simulink model "QDrone_Capture_IMU"  (R2019a)
settings: Solver=ode2  StartTime=0.0  StopTime=inf  FixedStep=0.001  RelTol=1e-3  EnableMultiTasking=on
InitFcn:
  | addpath(fullfile(fileparts(get_param('QDrone_Capture_IMU','FileName')),'capture_tool'));
model workspace (MAT data in the model file):
  target_system = 1
undefined symbols (not defined in the file or in its folder): HIL, qc_get_step_size
libraries: quarc_library x7
settings Model: SimulationMode=external  ExtModeTrigDuration=10000  Creator=dmadill  LastModifiedBy=user
settings SolverCC: PositivePriorityOrder=on
settings DataIOCC: LimitDataPoints=on  SaveFormat=Array  ReturnWorkspaceOutputs=off
settings OptimizationCC: LifeSpan=inf
settings DebuggingCC: SolverPrmCheckMsg=warning  SFUnexpectedBacktrackingDiag=warning  SFNoUnconditionalDefaultTransitionDiag=warning  SFExecutionAtInitializationDiag=none  ArithmeticOperatorsInVariantConditions=warning
settings HardwareCC: ProdBitPerLong=64  ProdLargestAtomicFloat=None  ProdHWDeviceType=Intel->x86-64
settings ModelReferenceCC: PropagateSignalLabelsOutOfModel=off
settings SFSimCC: SimUseLocalCustomCode=off
settings RTWCC: SystemTargetFile=quarc_linux_x64.tlc  TemplateMakefile=quarc_linux_x64_tmf  Description=QUARC Linux x64 Target  RTWUseLocalCustomCode=off
settings CodeAppCC: StateflowObjectComments=on
settings STFCustomTargetCC: TargetLibSuffix=.a  TargetPreCompLibLocation=C:\PROGRA~3\QUARC\lib\2019a\LINUX_~1\release  ConcurrentExecutionCompliant=on  SystemTargetFile=quarc_linux_x64.tlc
settings GRTTargetCC: TargetLibSuffix=.a  TargetPreCompLibLocation=C:\PROGRA~3\QUARC\lib\2019a\LINUX_~1\release  TargetLangStandard=C89/C90 (ANSI)  ParMdlRefBuildCompliant=off  CompOptLevelCompliant=off  CombineOutputUpdateFcns=off  MatFileLogging=off  CPPClassGenCompliant=off  GRTInterface=on  UseToolchainInfoCompliant=off  ExtMode=on  ExtModeMexFile=quarc_comm  ExtModeMexArgs='-w -d /tmp -uri %u', 'tcpip://192.168.2.52:17001?retries=10', 'tcpip://192.168.2.52:17000'
settings ConfigComp: CovMetricSettings=dw  CovHtmlReporting=on  CovSaveCumulativeToWorkspaceVar=on  CovSaveSingleToWorkspaceVar=on  CovExternalEMLEnable=off  CovSFcnEnable=off

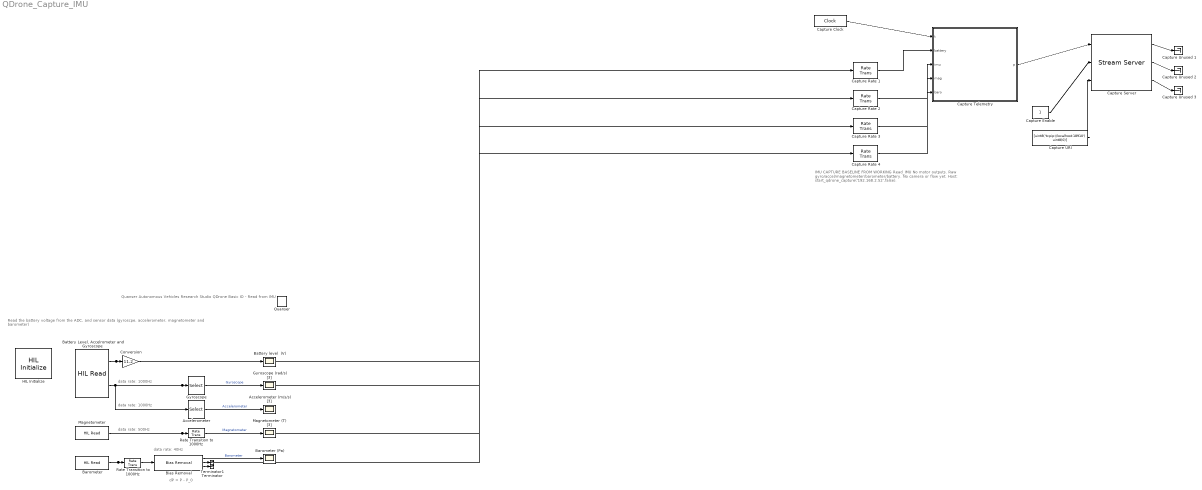
== system QDrone_Capture_IMU ==
  note: Quanser Autonomous Vehicles Research Studio
      | QDrone Basic IO - Read from IMU
  note: Read the battery voltage from the ADC, and sensor data (gyroscpe, accelerometer, magnetometer and barometer)
  note: data rate: 40Hz
  note: dP = P - P_0
  note: data rate: 500Hz
  note: data rate: 1000Hz
  note: data rate: 1000Hz
  note: IMU CAPTURE BASELINE FROM WORKING Read_IMU
      | No motor outputs. Raw gyro/accel/magnetometer/barometer/battery.
      | No camera or flow yet. Host: start_qdrone_capture('192.168.2.52',false).
  Accelerometer : Selector  InputPortWidth=6  IndexOptions=Index vector (dialog)  Indices=[4:6]  OutputSizes=1
  Accelerometer (m/s/s) [3] : Scope
  Barometer : quarc_library/Data Acquisition/Generic/Immediate I//O/HIL Read  Priority=1  object_name=HIL-1  analog_channels=[]  encoder_channels=[]  digital_channels=[]  other_channels=[9000]  sample_time=qc_get_step_size*25  active=on  vector_output=on  data_type_mode=Inherit via back propagation  encoder_data_type=double  digital_data_type=boolean
      settings: SourceProductName=The database C:\Users\user\AppData\Roaming\MathWorks\MATLAB\R2017a\slblocks_master.db is locked, or a table in the database is locked. (database is locked)
  Barometer (Pa) : Scope
  "Battery Level, Accelrometer and Gyroscope" : quarc_library/Data Acquisition/Generic/Immediate I//O/HIL Read  Priority=1  object_name=HIL-1  analog_channels=[4]  encoder_channels=[]  digital_channels=[]  other_channels=[3000:3002 4000:4002]  sample_time=qc_get_step_size  active=on  vector_output=on  data_type_mode=Inherit via back propagation  encoder_data_type=double  digital_data_type=boolean
      settings: SourceProductName=The database C:\Users\user\AppData\Roaming\MathWorks\MATLAB\R2017a\slblocks_master.db is locked, or a table in the database is locked. (database is locked)
  Battery level  (V) : Scope
  Bias Removal : quarc_library/Discrete/Bias Removal  start_time=0  end_time=2  switch_id=X  sample_time=qc_get_step_size
      settings: SourceProductName=QUARC Targets
  Capture Clock : DigitalClock  SampleTime=0.001
  Capture Enable : Constant
  Capture Rate {1..4} (4 alike) : RateTransition  OutPortSampleTime=0.001
  Capture Server : quarc_library/Communications/Basic/Stream Server  uri_source=External input port  uri=tcpip://remotehost:18000  apply_uri_to_all_configs=on  send_buffer_size=65536  receive_buffer_size=1024  byte_order=little endian (Intel - LSB first)  optimization=Minimum latency  send_options=Send all data  receive_options=Do not receive data  default_value=[0]  sample_time=0.001  active=on  implementation=Use blocking I/O in a separate thread  send_fifo_size=20000  receive_fifo_size=1000  send_priority=0  receive_priority=0  send_dimensions=off  receive_dimensions=off  max_dimensions=-1  data_type=Inherited via back propagation  type_expr=BusObject
  Capture Telemetry : MATLAB Function  TreatAsAtomicUnit=on
  Capture URI : Constant  Value=[uint8('tcpip://localhost:18910') uint8(0)]
  Capture Unused 1 : Terminator
  Capture Unused 2 : Terminator
  Capture Unused 3 : Terminator
  Conversion : Gain  Gain=11.2
  Gyroscope : Selector  InputPortWidth=6  IndexOptions=Index vector (dialog)  Indices=[1:3]  OutputSizes=1
  Gyroscope (rad/s) [3] : Scope
  HIL Initialize : quarc_library/Data Acquisition/Generic/Configuration/HIL Initialize  object_name=HIL-1  board_type=qdrone  board_number=0  board_options=gyro_fs=2000;gyro_rate=1000;gyro_os=4;accel_fs=16;accel_rate=400;accel_os=4;baro_os=4096  exclusive=off  active=on  hardware_clocks=[]  clock_modes=[]  initial_clock_frequencies=[]  set_clock_params_at_start=off  set_clock_params_at_switch_in=off  set_clock_frequencies_at_start=off  set_clock_frequencies_at_switch_in=off  analog_input_channels=[0:4]  analog_input_configurations=[]  analog_input_maximums=[3.3]  analog_input_minimums=[0]  set_analog_input_params_at_start=off  set_analog_input_params_at_switch_in=off  analog_output_channels=[]  analog_output_maximums=[]  analog_output_minimums=[]  initial_analog_outputs=[]  final_analog_outputs=[]  watchdog_analog_outputs=[]  set_analog_output_params_at_start=off  set_analog_output_params_at_switch_in=off  set_analog_outputs_at_start=off  set_analog_outputs_at_switch_in=off  set_analog_outputs_at_terminate=off  set_analog_outputs_at_switch_out=off  set_analog_outputs_on_watchdog=off  digital_input_channels=[]  digital_output_channels=[]  digital_output_configuration=[]  initial_digital_outputs=[0]  final_digital_outputs=[0]  watchdog_digital_outputs=[]  set_digital_output_params_at_start=off  set_digital_output_params_at_switch_in=off  set_digital_outputs_at_start=off  set_digital_outputs_at_switch_in=off  set_digital_outputs_at_terminate=off  set_digital_outputs_at_switch_out=off  set_digital_outputs_on_watchdog=off  encoder_channels=[]  quadrature=[4]  encoder_filter_frequency=50e6/1  initial_encoder_counts=[0]  set_encoder_params_at_start=off  set_encoder_params_at_switch_in=off  set_encoder_counts_at_start=off  set_encoder_counts_at_switch_in=off  pwm_channels=[]  pwm_modes=[4]  pwm_frequency=2000  pwm_configuration=[0]  pwm_alignment=[0]  pwm_polarity=[1]  pwm_leading_deadband=[]  pwm_trailing_deadband=[]  initial_pwm_outputs=[0]  final_pwm_outputs=[0]  watchdog_pwm_outputs=[0]  set_pwm_params_at_start=off  set_pwm_params_at_switch_in=off  set_pwm_outputs_at_start=off  set_pwm_outputs_at_switch_in=off  set_pwm_outputs_at_terminate=off  set_pwm_outputs_at_switch_out=off  set_pwm_outputs_on_watchdog=off  other_output_channels=[]  initial_other_outputs=[]  final_other_outputs=[]  watchdog_other_outputs=[]  set_other_outputs_at_start=off  set_other_outputs_at_switch_in=off  set_other_outputs_at_terminate=off  set_other_outputs_at_switch_out=off  set_other_outputs_on_watchdog=off
      settings: SourceProductName=The database C:\Users\user\AppData\Roaming\MathWorks\MATLAB\R2017a\slblocks_master.db is locked, or a table in the database is locked. (database is locked)
  Magnetometer : quarc_library/Data Acquisition/Generic/Immediate I//O/HIL Read  Priority=1  object_name=HIL-1  analog_channels=[]  encoder_channels=[]  digital_channels=[]  other_channels=[8000:8002]  sample_time=qc_get_step_size*2  active=on  vector_output=on  data_type_mode=Inherit via back propagation  encoder_data_type=double  digital_data_type=boolean
      settings: SourceProductName=The database C:\Users\user\AppData\Roaming\MathWorks\MATLAB\R2017a\slblocks_master.db is locked, or a table in the database is locked. (database is locked)
  Magnetometer (T) [3] : Scope
  Quanser : quarc_library/Logos/Quanser
  Rate Transition to 1000Hz : RateTransition
  Rate Transition to 1000Hz : RateTransition  OutPortSampleTime=qc_get_step_size
  Terminator : Terminator
  Terminator1 : Terminator
  wires:
  Accelerometer/1 -> Accelerometer (m/s/s) [3]/1  "Accelerometer"
  Bias Removal/3 -> Terminator/1
  Gyroscope/1 -> Gyroscope (rad/s) [3]/1  "Gyroscope"
  Barometer/1 -> Rate Transition to 1000Hz/1, Capture Rate 4/1
  Bias Removal/1 -> Barometer (Pa)/1  "Barometer"
  "Battery Level, Accelrometer and Gyroscope"/1 -> Conversion/1, Capture Rate 1/1
  Bias Removal/2 -> Terminator1/1
  Magnetometer/1 -> Rate Transition to 1000Hz/1, Capture Rate 3/1
  Rate Transition to 1000Hz/1 -> Magnetometer (T) [3]/1  "Magnetometer"
  Conversion/1 -> Battery level  (V)/1
  "Battery Level, Accelrometer and Gyroscope"/2 -> Capture Rate 2/1, Gyroscope/1, Accelerometer/1
  Rate Transition to 1000Hz/1 -> Bias Removal/1
  Capture Clock/1 -> Capture Telemetry/1(t)
  Capture Rate 1/1 -> Capture Telemetry/2(battery)
  Capture Rate 2/1 -> Capture Telemetry/3(imu)
  Capture Rate 3/1 -> Capture Telemetry/4(mag)
  Capture Rate 4/1 -> Capture Telemetry/5(baro)
  Capture Telemetry/1(p) -> Capture Server/1
  Capture Enable/1 -> Capture Server/2
  Capture URI/1 -> Capture Server/3
  Capture Server/1 -> Capture Unused 1/1
  Capture Server/2 -> Capture Unused 2/1
  Capture Server/3 -> Capture Unused 3/1

== matlab function QDrone_Capture_IMU/Capture Telemetry ==
  data: t input; p output; battery input; imu input; mag input; baro input
function p=run(t,battery,imu,mag,baro)
%#codegen
p=[51234567;1;round(t/0.001);t;nan(4,1);battery;imu(:);mag(:);baro;NaN;zeros(8,1);0;0];
end
